simulink model "Exp6_FuzzyGA_ELD_Sim"  (R2025b)
settings: Solver=FixedStepDiscrete  StartTime=0  StopTime=199  FixedStep=1  RelTol=1e-3
model workspace (MAT data in the model file):
  Exp6_B = [1.7e-05  1.2e-05  7e-06  -1e-06  -5e-06  -2e-06; 1.2e-05  1.4e-05  9e-06  1e-06  -6e-06  -1e-06; 7e-06  9e-06  3.1e-05  0  -1e-05  -6e-06; -1e-06  1e-06  0  2.4e-05  -6e-06  -8e-06; -5e-06  -6e-06  -1e-05  -6e-06  0.000129  -2e-06; -2e-06  -1e-06  -6e-06  -8e-06  -2e-06  0.00015]
  Exp6_B0 = [-0.0003908 -0.0001297 0.0007047 5.91e-05 0.0002161 -0.0006635]
  Exp6_B00 = 0.56
  Exp6_G = 200
  Exp6_IC = [0.8; 0.05; 0.102]
  Exp6_N = 30
  Exp6_PD = 800
  Exp6_a = [240; 200; 220; 200; 220; 190]
  Exp6_b = [7; 10; 8.5; 11; 10.5; 12]
  Exp6_c = [0.007; 0.0095; 0.009; 0.009; 0.008; 0.0075]
  Exp6_fis : mamfis (value not decoded)
  Exp6_prm.a = [240 200 220 200 220 190]
  Exp6_prm.b = [7 10 8.5 11 10.5 12]
  Exp6_prm.c = [0.007 0.0095 0.009 0.009 0.008 0.0075]
  Exp6_prm.B = [1.7e-05  1.2e-05  7e-06  -1e-06  -5e-06  -2e-06; 1.2e-05  1.4e-05  9e-06  1e-06  -6e-06  -1e-06; 7e-06  9e-06  3.1e-05  0  -1e-05  -6e-06; -1e-06  1e-06  0  2.4e-05  -6e-06  -8e-06; -5e-06  -6e-06  -1e-05  -6e-06  0.000129  -2e-06; -2e-06  -1e-06  -6e-06  -8e-06  -2e-06  0.00015]
  Exp6_prm.B0 = [-0.0003908 -0.0001297 0.0007047 5.91e-05 0.0002161 -0.0006635]
  Exp6_prm.B00 = 0.56
  Exp6_prm.PD = 800
  Exp6_prm.POZ = [210  240  350  380; 90  110  140  160; 150  170  210  240; 80  90  110  120; 90  110  140  150; 75  85  100  105]
  Exp6_prm.lo = [320 80 100 60 100 50]
  Exp6_prm.hi = [500 200 265 150 200 120]
  Exp6_prm.usePOZ = 1
  Exp6_prm.kPen = 1000
  Exp6_prm.caseNo = 2
  Exp6_seed = 1
  Exp6_useFuzzy = 1
libraries: fuzblock x1
settings Model: Creator=mithu  LastModifiedBy=mithu

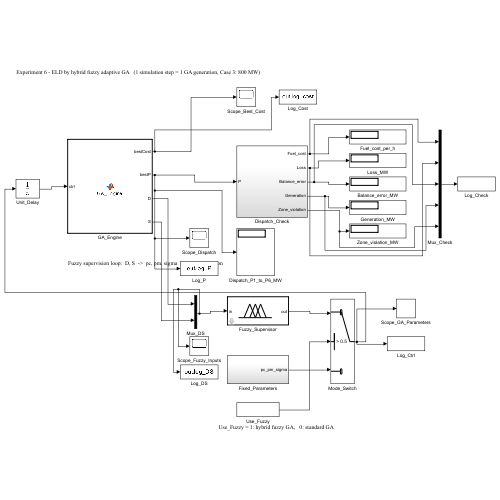
[thumbnail: Simulink's stored preview of the top-level diagram]
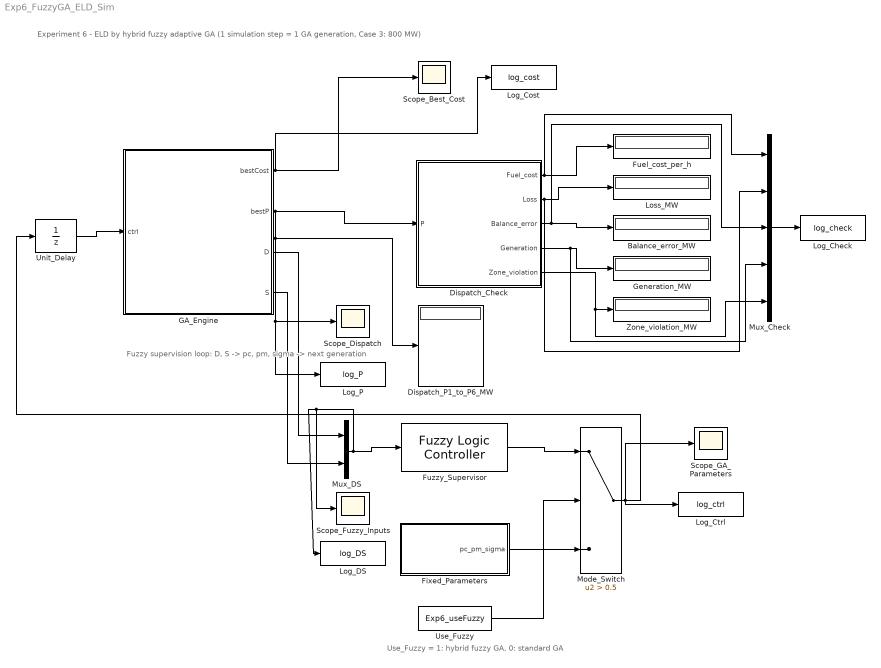
== system Exp6_FuzzyGA_ELD_Sim ==
  note: Experiment 6 - ELD by hybrid fuzzy adaptive GA (1 simulation step = 1 GA generation, Case 3: 800 MW)
  note: Fuzzy supervision loop: D, S -> pc, pm, sigma -> next generation
  note: Use_Fuzzy = 1: hybrid fuzzy GA, 0: standard GA
  Balance_error_MW : Display
  Dispatch_Check : Subsystem
  Dispatch_P1_to_P6_MW : Display
  Fixed_Parameters : Subsystem
  Fuel_cost_per_h : Display
  Fuzzy_Supervisor : fuzblock/Fuzzy Logic  Controller  FIS=Exp6_fis  OutputSampleNumber=101  DataType=double  UseLookupTable=off  NumBreakpoints=10  FuzzifiedInputs=off  RuleFiringStrengths=off  RuleOutputs=off  AggregatedOutputs=off  SimulateUsing=Interpreted execution  OutOfRangeInputValueMessage=none  NoRuleFiredMessage=none  EmptyOutputFuzzySetMessage=none
  GA_Engine : MATLAB Function  TreatAsAtomicUnit=on
  Generation_MW : Display
  Log_Check : ToWorkspace  VariableName=log_check  SampleTime=-1
  Log_Cost : ToWorkspace  VariableName=log_cost  SampleTime=-1
  Log_Ctrl : ToWorkspace  VariableName=log_ctrl  SampleTime=-1
  Log_DS : ToWorkspace  VariableName=log_DS  SampleTime=-1
  Log_P : ToWorkspace  VariableName=log_P  SampleTime=-1
  Loss_MW : Display
  Mode_Switch : Switch  Criteria=u2 > Threshold  Threshold=0.5  SaturateOnIntegerOverflow=off  InputSameDT=off
  Mux_Check : Mux  Inputs=5
  Mux_DS : Mux  Inputs=2
  Scope_Best_Cost : Scope
  Scope_Dispatch : Scope
  Scope_Fuzzy_Inputs : Scope
  Scope_GA_Parameters : Scope
  Unit_Delay : UnitDelay  InitialCondition=Exp6_IC  HasFrameUpgradeWarning=on
  Use_Fuzzy : Constant  Value=Exp6_useFuzzy
  Zone_violation_MW : Display
  wires:
  Unit_Delay/1 -> GA_Engine/1(ctrl)
  GA_Engine/1(bestCost) -> Scope_Best_Cost/1, Log_Cost/1
  GA_Engine/2(bestP) -> Log_P/1, Scope_Dispatch/1, Dispatch_P1_to_P6_MW/1, Dispatch_Check/1(P)
  GA_Engine/3(D) -> Mux_DS/1
  GA_Engine/4(S) -> Mux_DS/2
  Mux_DS/1 -> Scope_Fuzzy_Inputs/1, Log_DS/1, Fuzzy_Supervisor/1
  Fuzzy_Supervisor/1 -> Mode_Switch/1
  Use_Fuzzy/1 -> Mode_Switch/2
  Fixed_Parameters/1(pc_pm_sigma) -> Mode_Switch/3
  Mode_Switch/1 -> Unit_Delay/1, Scope_GA_Parameters/1, Log_Ctrl/1
  Dispatch_Check/1(Fuel_cost) -> Fuel_cost_per_h/1, Mux_Check/1
  Dispatch_Check/2(Loss) -> Loss_MW/1, Mux_Check/2
  Dispatch_Check/3(Balance_error) -> Balance_error_MW/1, Mux_Check/3
  Dispatch_Check/4(Generation) -> Generation_MW/1, Mux_Check/4
  Dispatch_Check/5(Zone_violation) -> Zone_violation_MW/1, Mux_Check/5
  Mux_Check/1 -> Log_Check/1

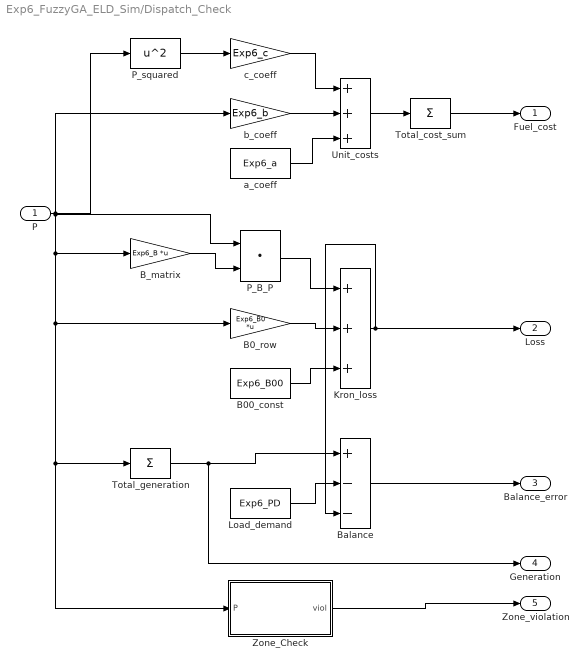
== system Exp6_FuzzyGA_ELD_Sim/Dispatch_Check ==
  P : Inport
  B00_const : Constant  Value=Exp6_B00
  B0_row : Gain  Gain=Exp6_B0  Multiplication=Matrix(K*u)
  B_matrix : Gain  Gain=Exp6_B  Multiplication=Matrix(K*u)
  Balance : Sum  Inputs=+--
  Kron_loss : Sum  Inputs=+++
  Load_demand : Constant  Value=Exp6_PD
  P_B_P : DotProduct  OutDataTypeStr=Inherit: Inherit via internal rule
  P_squared : Math  Operator=square
  Total_cost_sum : Sum  Inputs=+
  Total_generation : Sum  Inputs=+
  Unit_costs : Sum  Inputs=+++
  Zone_Check : MATLAB Function  TreatAsAtomicUnit=on
  a_coeff : Constant  Value=Exp6_a
  b_coeff : Gain  Gain=Exp6_b
  c_coeff : Gain  Gain=Exp6_c
  Fuel_cost : Outport
  Loss : Outport  Port=2
  Balance_error : Outport  Port=3
  Generation : Outport  Port=4
  Zone_violation : Outport  Port=5
  wires:
  P/1 -> Total_generation/1, Zone_Check/1(P), B0_row/1, B_matrix/1, P_B_P/1, P_squared/1, b_coeff/1
  P_squared/1 -> c_coeff/1
  c_coeff/1 -> Unit_costs/1
  b_coeff/1 -> Unit_costs/2
  a_coeff/1 -> Unit_costs/3
  Unit_costs/1 -> Total_cost_sum/1
  Total_cost_sum/1 -> Fuel_cost/1
  B_matrix/1 -> P_B_P/2
  P_B_P/1 -> Kron_loss/1
  B0_row/1 -> Kron_loss/2
  B00_const/1 -> Kron_loss/3
  Kron_loss/1 -> Loss/1, Balance/3
  Total_generation/1 -> Balance/1, Generation/1
  Load_demand/1 -> Balance/2
  Balance/1 -> Balance_error/1
  Zone_Check/1(viol) -> Zone_violation/1

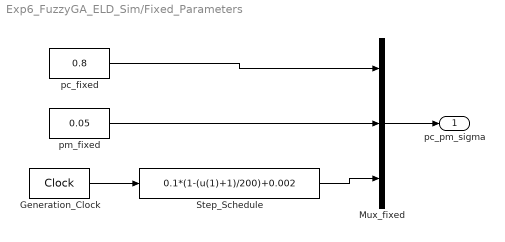
== system Exp6_FuzzyGA_ELD_Sim/Fixed_Parameters ==
  Generation_Clock : DigitalClock
  Mux_fixed : Mux  Inputs=3
  Step_Schedule : Fcn  Expr=0.1*(1-(u(1)+1)/200)+0.002
  pc_fixed : Constant  Value=0.8
  pm_fixed : Constant  Value=0.05
  pc_pm_sigma : Outport
  wires:
  pc_fixed/1 -> Mux_fixed/1
  pm_fixed/1 -> Mux_fixed/2
  Generation_Clock/1 -> Step_Schedule/1
  Step_Schedule/1 -> Mux_fixed/3
  Mux_fixed/1 -> pc_pm_sigma/1

== matlab function Exp6_FuzzyGA_ELD_Sim/Dispatch_Check/Zone_Check ==
  data: P input; viol output; Exp6_prm parameter
function viol = Zone_Check(P, Exp6_prm)
% depth (MW) of operation inside prohibited zones, 0 = all units in allowed segments
[~, ~, ~, ~, viol] = eld_evaluate(P.', Exp6_prm);
end

== matlab function Exp6_FuzzyGA_ELD_Sim/GA_Engine ==
  data: ctrl input size=3; bestCost output; bestP output; D output; S output; Exp6_prm parameter; Exp6_N parameter; Exp6_seed parameter
function [bestCost, bestP, D, S] = GA_Engine(ctrl, Exp6_prm, Exp6_N, Exp6_seed)
% One call = one generation of the real-coded GA.
% ctrl = [pc; pm; sigma] chosen by the fuzzy supervisor (or the fixed values)
% for this generation. Outputs describe the population after the generation.
prm = Exp6_prm;  N = Exp6_N;
persistent pop fit best stall
if isempty(pop)
    rng(Exp6_seed, 'twister');
    range = prm.hi - prm.lo;
    pop = eld_repair(prm.lo + rand(N, numel(range)).*range, prm);
    fit = eld_evaluate(pop, prm);
    best = min(fit);   stall = 0;
end
[pop, fit] = ga_generation(pop, fit, ctrl(1), ctrl(2), ctrl(3), prm);
[bestCost, ib] = min(fit);
if bestCost < best - 1e-3, stall = 0; else, stall = stall + 1; end
best = min(best, bestCost);
bestP = pop(ib, :).';
D = pop_diversity(pop, prm);
S = min(stall/20, 1);
end
